simulink model "Shaddad_Companion"  (R2026b)
undefined symbols (not defined in the file): P, Ts
settings Model: Creator=aomar  LastModifiedBy=aomar

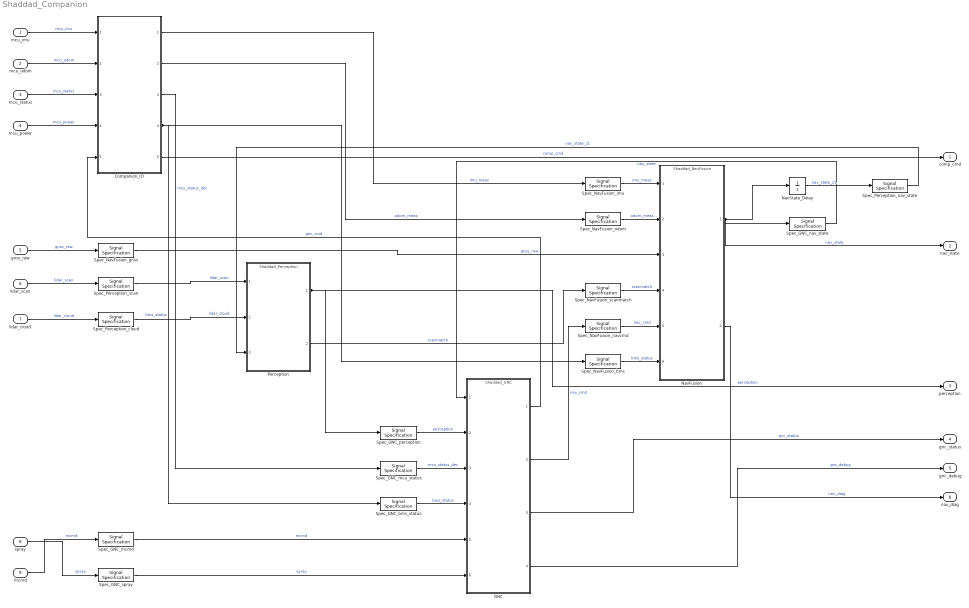
== system Shaddad_Companion ==
  mcu_imu : Inport  OutDataTypeStr=Bus: Bus_CanFrame64  SampleTime=Ts.imu  BusOutputAsStruct=on
  mcu_odom : Inport  Port=2  OutDataTypeStr=Bus: Bus_CanFrame64  SampleTime=Ts.ctrl  BusOutputAsStruct=on
  mcu_status : Inport  Port=3  OutDataTypeStr=Bus: Bus_CanFrame64  SampleTime=Ts.comm  BusOutputAsStruct=on
  mcu_power : Inport  Port=4  OutDataTypeStr=Bus: Bus_CanFrame64  SampleTime=Ts.hk  BusOutputAsStruct=on
  gnss_raw : Inport  Port=5  OutDataTypeStr=Bus: Bus_GnssRaw  SampleTime=Ts.hk  BusOutputAsStruct=on
  lidar_scan : Inport  Port=6  OutDataTypeStr=Bus: Bus_LidarScanRaw  SampleTime=Ts.hk  BusOutputAsStruct=on
  lidar_cloud : Inport  Port=7  OutDataTypeStr=Bus: Bus_LidarCloudRaw  SampleTime=Ts.hk  BusOutputAsStruct=on
  spray : Inport  Port=8  OutDataTypeStr=Bus: Bus_SprayDemand  SampleTime=Ts.hk  BusOutputAsStruct=on
  mcmd : Inport  Port=9  OutDataTypeStr=Bus: Bus_MissionCmd  SampleTime=Ts.gnc_status  BusOutputAsStruct=on
  Companion_IO : Subsystem  ReferencedSubsystem=companion_io
  GNC : ModelReference  ModelNameDialog=Shaddad_GNC  SimulationMode=Normal  ModelReferenceVersion=1.1
  NavFusion : ModelReference  ModelNameDialog=Shaddad_NavFusion  SimulationMode=Normal  ModelReferenceVersion=1.1
  NavState_Delay : UnitDelay  InitialCondition=P.ic.Bus_NavState  SampleTime=Ts.nav
  Perception : ModelReference  ModelNameDialog=Shaddad_Perception  SimulationMode=Normal  ModelReferenceVersion=1.1
  Spec_GNC_bms_status : SignalSpecification  OutDataTypeStr=Bus: Bus_BmsStatus  SampleTime=Ts.hk  BusOutputAsStruct=on
  Spec_GNC_mcmd : SignalSpecification  OutDataTypeStr=Bus: Bus_MissionCmd  SampleTime=Ts.gnc_status  BusOutputAsStruct=on
  Spec_GNC_mcu_status : SignalSpecification  OutDataTypeStr=Bus: Bus_McuStatus  SampleTime=Ts.comm  BusOutputAsStruct=on
  Spec_GNC_nav_state : SignalSpecification  OutDataTypeStr=Bus: Bus_NavState  SampleTime=Ts.ctrl  BusOutputAsStruct=on
  Spec_GNC_perception : SignalSpecification  OutDataTypeStr=Bus: Bus_Perception  SampleTime=Ts.hk  BusOutputAsStruct=on
  Spec_GNC_spray : SignalSpecification  OutDataTypeStr=Bus: Bus_SprayDemand  SampleTime=Ts.hk  BusOutputAsStruct=on
  Spec_NavFusion_bms : SignalSpecification  OutDataTypeStr=Bus: Bus_BmsStatus  SampleTime=Ts.hk  BusOutputAsStruct=on
  Spec_NavFusion_gnss : SignalSpecification  OutDataTypeStr=Bus: Bus_GnssRaw  SampleTime=Ts.hk  BusOutputAsStruct=on
  Spec_NavFusion_imu : SignalSpecification  OutDataTypeStr=Bus: Bus_ImuMeas  SampleTime=Ts.imu  BusOutputAsStruct=on
  Spec_NavFusion_navcmd : SignalSpecification  OutDataTypeStr=Bus: Bus_NavCmd  SampleTime=Ts.comm  BusOutputAsStruct=on
  Spec_NavFusion_odom : SignalSpecification  OutDataTypeStr=Bus: Bus_OdomMeas  SampleTime=Ts.ctrl  BusOutputAsStruct=on
  Spec_NavFusion_scanmatch : SignalSpecification  OutDataTypeStr=Bus: Bus_ScanMatchMeas  SampleTime=Ts.gnc_status  BusOutputAsStruct=on
  Spec_Perception_cloud : SignalSpecification  OutDataTypeStr=Bus: Bus_LidarCloudRaw  SampleTime=Ts.hk  BusOutputAsStruct=on
  Spec_Perception_nav_state : SignalSpecification  OutDataTypeStr=Bus: Bus_NavState  SampleTime=Ts.ctrl  BusOutputAsStruct=on
  Spec_Perception_scan : SignalSpecification  OutDataTypeStr=Bus: Bus_LidarScanRaw  SampleTime=Ts.hk  BusOutputAsStruct=on
  comp_cmd : Outport  OutDataTypeStr=Bus: Bus_CanFrame64  SampleTime=Ts.comm  BusOutputAsStruct=on
  nav_state : Outport  Port=2  OutDataTypeStr=Bus: Bus_NavState  SampleTime=Ts.ctrl  BusOutputAsStruct=on
  perception : Outport  Port=3  OutDataTypeStr=Bus: Bus_Perception  SampleTime=Ts.hk  BusOutputAsStruct=on
  gnc_status : Outport  Port=4  OutDataTypeStr=Bus: Bus_GncStatus  SampleTime=Ts.gnc_status  BusOutputAsStruct=on
  gnc_debug : Outport  Port=5  OutDataTypeStr=Bus: Bus_GncDebug  SampleTime=Ts.comm  BusOutputAsStruct=on
  nav_diag : Outport  Port=6  OutDataTypeStr=Bus: Bus_NavDiag  SampleTime=Ts.ctrl  BusOutputAsStruct=on
  wires:
  mcu_imu/1 -> Companion_IO/1  "mcu_imu"
  mcu_odom/1 -> Companion_IO/2  "mcu_odom"
  mcu_status/1 -> Companion_IO/3  "mcu_status"
  mcu_power/1 -> Companion_IO/4  "mcu_power"
  gnss_raw/1 -> Spec_NavFusion_gnss/1  "gnss_raw"
  lidar_scan/1 -> Spec_Perception_scan/1  "lidar_scan"
  lidar_cloud/1 -> Spec_Perception_cloud/1  "lidar_cloud"
  spray/1 -> Spec_GNC_spray/1  "spray"
  mcmd/1 -> Spec_GNC_mcmd/1  "mcmd"
  Spec_NavFusion_gnss/1 -> NavFusion/3  "gnss_raw"
  Spec_Perception_scan/1 -> Perception/1  "lidar_scan"
  Spec_Perception_cloud/1 -> Perception/2  "lidar_cloud"
  Spec_GNC_mcmd/1 -> GNC/5  "mcmd"
  Spec_GNC_spray/1 -> GNC/6  "spray"
  Companion_IO/1 -> Spec_NavFusion_imu/1  "imu_meas"
  Companion_IO/2 -> Spec_NavFusion_odom/1  "odom_meas"
  Companion_IO/3 -> Spec_GNC_mcu_status/1  "mcu_status_dec"
  Companion_IO/4 -> Spec_GNC_bms_status/1, Spec_NavFusion_bms/1  "bms_status"
  Companion_IO/5 -> comp_cmd/1  "comp_cmd"
  Perception/1 -> Spec_GNC_perception/1, perception/1  "perception"
  Perception/2 -> Spec_NavFusion_scanmatch/1  "scanmatch"
  Spec_GNC_perception/1 -> GNC/2  "perception"
  Spec_GNC_mcu_status/1 -> GNC/3  "mcu_status_dec"
  Spec_GNC_bms_status/1 -> GNC/4  "bms_status"
  GNC/1 -> Companion_IO/5  "gnc_cmd"
  GNC/2 -> Spec_NavFusion_navcmd/1  "nav_cmd"
  GNC/3 -> gnc_status/1  "gnc_status"
  GNC/4 -> gnc_debug/1  "gnc_debug"
  Spec_NavFusion_imu/1 -> NavFusion/1  "imu_meas"
  Spec_NavFusion_odom/1 -> NavFusion/2  "odom_meas"
  Spec_NavFusion_scanmatch/1 -> NavFusion/4  "scanmatch"
  Spec_NavFusion_navcmd/1 -> NavFusion/5  "nav_cmd"
  Spec_NavFusion_bms/1 -> NavFusion/6  "bms_status"
  NavFusion/1 -> NavState_Delay/1, nav_state/1, Spec_GNC_nav_state/1  "nav_state"
  NavFusion/2 -> nav_diag/1  "nav_diag"
  NavState_Delay/1 -> Spec_Perception_nav_state/1  "nav_state_z1"
  Spec_GNC_nav_state/1 -> GNC/1  "nav_state"
  Spec_Perception_nav_state/1 -> Perception/3  "nav_state_z1"
